simulink model "GeradorDADOS"  (R2023b)
settings: Solver=FixedStepAuto  StartTime=0.0  StopTime=(1500-1)*Ts  FixedStep=Ts/100  RelTol=1e-3
values from neighbouring files (symbols this model uses):
  C = 0.000143    [IdentificacaoARXboost.m]
  Ts = 5.0e-5    (= 5e-05)    [IdentificacaoARXboost.m]
  Vs = 30    [IdentificacaoARXboost.m]
libraries: spsSeriesRLCBranchLib x3, spsCurrentMeasurementLib x1, spsDiodeLib x1, spsDCVoltageSourceLib x1, spsGroundLib x1, spsMosfetLib x1, commseqgen3 x1, spsVoltageMeasurementLib x1, sps_lib x1
settings Model: Creator=Raphael Teixeira  LastModifiedBy=luisf
settings RTWCC: GPUComputeCapability=5.0

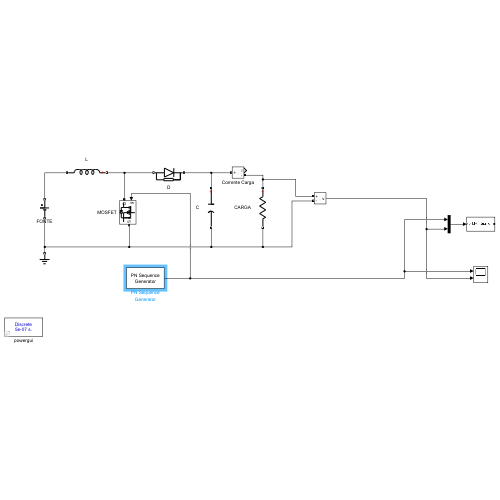
[thumbnail: Simulink's stored preview of the top-level diagram]
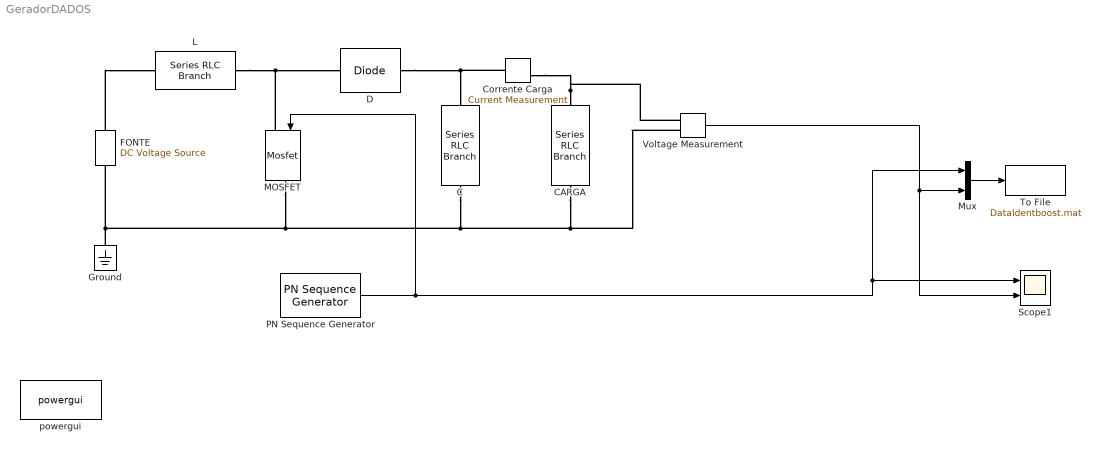
== system GeradorDADOS ==
  C : spsSeriesRLCBranchLib/Series RLC Branch  LConnTagsString=__new0  RConnTagsString=__new0  BranchType=C  Resistance=1  Inductance=1e-3  SetiL0=off  InitialCurrent=0  Capacitance=C  Setx0=off  InitialVoltage=0  Measurements=None
  CARGA : spsSeriesRLCBranchLib/Series RLC Branch  LConnTagsString=__new0  RConnTagsString=__new0  BranchType=R  Resistance=15  Inductance=1e-3  SetiL0=off  InitialCurrent=0  Capacitance=1e-6  Setx0=off  InitialVoltage=0  Measurements=None
  Corrente Carga : spsCurrentMeasurementLib/Current Measurement  PhasorSimulation=off  OutputType=Complex  PSBequivalent=0
  D : spsDiodeLib/Diode  Ron=0.001  Lon=0  Vf=1.7  IC=0  UseSnubber=0  Rs=500  Cs=250e-9  Measurements=off
  FONTE : spsDCVoltageSourceLib/DC Voltage Source  Amplitude=Vs  Measurements=None
  Ground : spsGroundLib/Ground  LConnTagsString=a
  L : spsSeriesRLCBranchLib/Series RLC Branch  LConnTagsString=__new0  RConnTagsString=__new0  BranchType=L  Resistance=1  Inductance=0.00056  SetiL0=off  InitialCurrent=0  Capacitance=1e-6  Setx0=off  InitialVoltage=0  Measurements=None
  MOSFET : spsMosfetLib/Mosfet  Ron=0.1  Lon=0  Rd=0.01  Vfd=0  IC=0  Rs=1e5  Cs=inf  Measurements=off
  Mux : Mux  Inputs=2
  PN Sequence Generator : commseqgen3/PN Sequence Generator  poly=[10 7 0]  ini_sta=ones(1, 10)  outBitMaskSource=Dialog parameter  shift=0  outVarSiz=off  maxOutSizeMode=Dialog parameter  maxOutSize=[10 1]  Ts=Ts  sampPerFrame=1  reset=off  bitPackedOutputs=off  outDataType=double  numPackedBits=8  bitPackDataSigned=off  bitPackedOutDType=double
  Scope1 : Scope  NumInputPorts=2
  To File : ToFile  Filename=DataIdentboost.mat  MatrixName=DadosBoost  SampleTime=Ts
  Voltage Measurement : spsVoltageMeasurementLib/Voltage Measurement  PhasorSimulation=off  OutputType=Complex  PSBequivalent=0
  powergui : sps_lib/powergui  Priority=1  SimulationMode=Discrete  SampleTime=Ts/100  frequency=60  Iterations=50  frequencyindice=0  Pbase=100e6  ErrMax=1e-4  UnitsV=kV  UnitsW=MW  buscounter=0  FunctionMessages=off  echomessages=off  EnableUseOfTLC=off  CurrentSourceSwitches=off  DisableSnubberDevices=off  DisableRonSwitches=off  DisableVfSwitches=off  DisplayEquations=off  AutomaticDiscreteSolvers=off  SolverType=Tustin/Backward Euler (TBE)  Interpol=off  ExternalGateDelay=off  methode=off  Ts=100  x0status=blocks  SPID=on  SwTol=0  HookPort=off  NonlinearTolerance=1e-4  nMaxIteration=100  ContinueOnMaxIteration=off  RestoreLinks=warning  ResistiveCurrentMeasurement=off  Frange=[0:2:500]  Ylog=off  Xlog=on  ShowGrid=off  save=off  variable=ZData  structure=0  ZoomFFT=off  StartTime=0.0  cycles=1  DisplayStyle=1  fundamental=60  FreqAxis=off  MaxFrequency=1000  frequencyindicesteady=1  RmsSteady=1  display=off
  wires:
  PN Sequence Generator/1 -> MOSFET/1, Scope1/1, Mux/1
  Voltage Measurement/1 -> Scope1/2, Mux/2
  Mux/1 -> To File/1
  connections:
  CARGA/RConn1 -- Voltage Measurement/LConn2 -- C/RConn1 -- MOSFET/RConn1 -- FONTE/LConn1 -- Ground/LConn1
  L/LConn1 -- MOSFET/LConn1 -- D/LConn1
  D/RConn1 -- Corrente Carga/LConn1 -- C/LConn1
  CARGA/LConn1 -- Voltage Measurement/LConn1 -- Corrente Carga/RConn1
  FONTE/RConn1 -- L/RConn1
